simulink model "ThermalLoop_draft3"  (R2024b)
settings: Solver=VariableStepAuto  StartTime=0.0  StopTime=2600
model workspace (MAT data in the model file):
  HX_HX = 500
  Kpipes = 14
  PumpHeat = 50
  TM_pipe = 50
libraries: fl_lib x28, nesl_utility x18, SimscapeFluids_lib x18, simulink x1
(part 1 of 2)
settings Model: SimulationMode=accelerator  Creator=Matthew Whetham  LastModifiedBy=Matthew Whetham

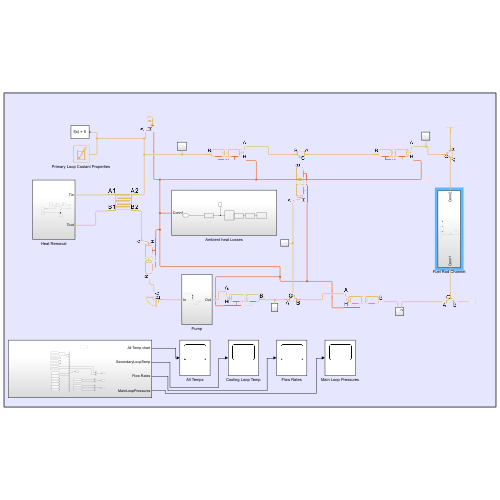
[thumbnail: Simulink's stored preview of the top-level diagram]
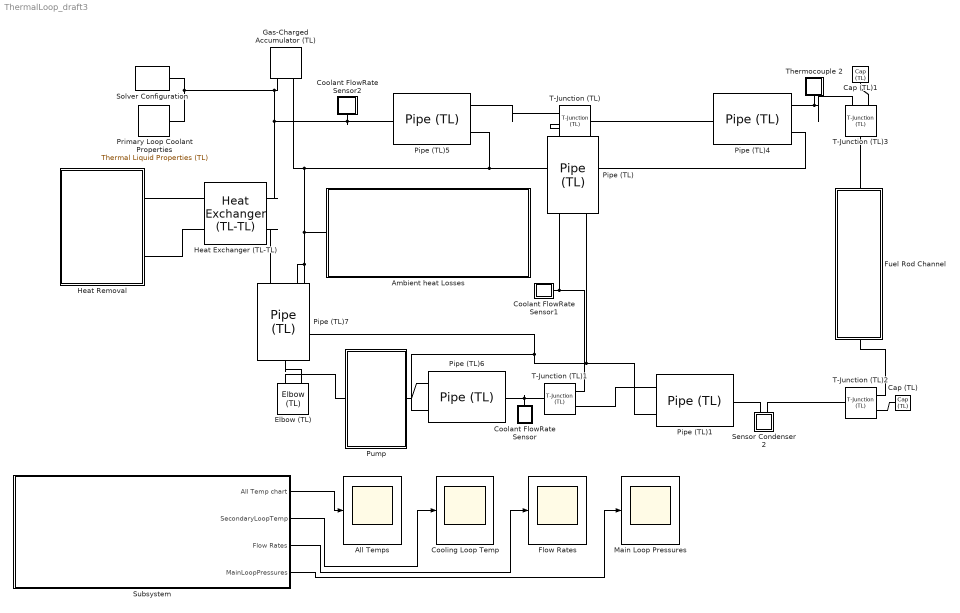
== system ThermalLoop_draft3 ==
  All Temps : Scope
  Ambient heat Losses : Subsystem
  Cap (TL) : fl_lib/Thermal Liquid/Elements/Cap (TL)  p_specify=off  p_priority=None  p=0.101325 MPa  p_nominal_specify=off  p_nominal_value=1  p_nominal_unit=MPa  T_specify=on  T_priority=Low  T=297.15 K  T_nominal_specify=off  T_nominal_value=1  T_nominal_unit=K
      settings: InternalSimscapePortConfiguration="{\"Bottom\":[],\"Left\":[{\"id\":\"A\",\"label\":\"\",\"type\":\"foundation.thermal_liquid.thermal_liquid\"}],\"Right\":[],\"Top\":[]}"
  Cap (TL)1 : fl_lib/Thermal Liquid/Elements/Cap (TL)  p_specify=off  p_priority=None  p=0.101325 MPa  p_nominal_specify=off  p_nominal_value=1  p_nominal_unit=MPa  T_specify=on  T_priority=None  T=297.15 K  T_nominal_specify=off  T_nominal_value=1  T_nominal_unit=K
      settings: InternalSimscapePortConfiguration="{\"Bottom\":[],\"Left\":[{\"id\":\"A\",\"label\":\"\",\"type\":\"foundation.thermal_liquid.thermal_liquid\"}],\"Right\":[],\"Top\":[]}"
  Coolant FlowRate Sensor : Subsystem
  Coolant FlowRate Sensor1 : Subsystem
  Coolant FlowRate Sensor2 : Subsystem
  Cooling Loop Temp : Scope
  Elbow (TL) : SimscapeFluids_lib/Thermal Liquid/Pipes & Fittings/Elbow (TL)  elbow_type=fluids.thermal_liquid.pipes_fittings.enum.ElbowType.Smooth  diameter_elbow=1.6 in  angle_elbow=90 deg  Re_c=150
      settings: InternalSimscapePortConfiguration="{\"Bottom\":[],\"Left\":[{\"id\":\"A\",\"label\":\"A\",\"type\":\"foundation.thermal_liquid.thermal_liquid\"}],\"Right\":[],\"Top\":[{\"id\":\"B\",\"label\":\"B\",\"type\":\"foundation.thermal_liquid.thermal_liquid\"}]}"
  Flow Rates : Scope
  Fuel Rod Channel : Subsystem
      settings: PortSchema="{\"entries\":[{\"content\":{\"sides\":[{\"content\":{},\"type\":\"ConnectorPlacement.EquallySpacedRectSide\",\"uuid\":\"06a059a3-807c-451a-afc8-2a90bcad8c1c\"},{\"content\":{\"side\":\"RIGHT\"},\"type\":\"ConnectorPlacement.EquallySpacedRectSide\",\"uuid\":\"c804ba08-1832-4016-bf14-7550ffa2d914\"},{\"content\":{\"connectorIds\":[\"LConn1\"],\"side\":\"TOP\"},\"type\":\"ConnectorPlacement.EquallySpacedRectSide\",\"uuid\":\"1e965a20-d254-4a65-95af-9e712761d911\"},{\"content\":{\"connectorIds\":[\"RConn1\"],\"side\":\"BOTTOM\"},\"type\":\"ConnectorPlacement.EquallySpacedRectSide\",\"uuid\":\"83471166-a379-4b82-b772-802eda07252c\"}]},\"type\":\"ConnectorPlacement.EquallySpacedConnector\",\"uuid\":\"06615f34-1427-44b4-a4dd-e60277b52231\"}],\"packageUris\":[\"http://schema.mathworks.com/mf0/Connector/R2020b\"],\"version\":\"1.0\"}"
  Gas-Charged Accumulator (TL) : SimscapeFluids_lib/Thermal Liquid/Tanks & Accumulators/Gas-Charged Accumulator (TL)  capacity=0.2 l  dead_volume=0.145 l  p_precharge_gauge=1 bar  k_sh=1.4  area=1.76 in^2  stiff_coeff=1e4 MPa/m^3  damping_coeff=1e4 MPa*s/m^6  liquid_volume_specify=off  liquid_volume_priority=High  liquid_volume=5e-3 m^3  liquid_volume_nominal_specify=off  liquid_volume_nominal_value=1  liquid_volume_nominal_unit=m^3  liquid_mass_specify=off  liquid_mass_priority=None  liquid_mass=5 kg  liquid_mass_nominal_specify=off  liquid_mass_nominal_value=1  liquid_mass_nominal_unit=kg  p_I_specify=off  p_I_priority=None  p_I=0.101325 MPa  p_I_nominal_specify=off  p_I_nominal_value=1  p_I_nominal_unit=MPa  T_I_specify=on  T_I_priority=Low  T_I=23 degC  T_I_nominal_specify=off  T_I_nominal_value=1  T_I_nominal_unit=K
      settings: InternalSimscapePortConfiguration="{\"Bottom\":[],\"Left\":[],\"Right\":[{\"id\":\"A\",\"label\":\"A\",\"type\":\"foundation.thermal_liquid.thermal_liquid\"},{\"id\":\"H\",\"label\":\"H\",\"type\":\"foundation.thermal.thermal\"}],\"Top\":[]}"
  Heat Exchanger (TL-TL) : SimscapeFluids_lib/Heat Exchangers/Thermal Liquid/Heat Exchanger (TL-TL)  hex_type=fluids.heat_exchangers.enum.FlowArrangement.ShellTube  shell_num=1  cross_type=fluids.heat_exchangers.enum.CrossFlowArrangementTLTL.MixedMixed  NTU_TLU=[.5, 1, 2, 3, 4, 5]  CR_TLU=[0, .25, .5, .75, 1]  eff_TLU=[.3, .3, .3, .3, .3; .6, .55, .5, .47, .43; .85, .76, .68, .61, .55; .94, .83, .72, .65, .58; .98, .86, .75, .66, .58; .99, .86, .75, .66, .58]  wall_thermal_dynamics=false  thermal_mass_wall=447 J/K  R_wall=1.6e-5 K/W  min_flow_area_1=1 m^2  Dh_press_1=0.1 m  liquid_volume_1=0.01 m^3  Re_lam_1=2000  Re_tur_1=4000  pressure_loss_spec_1=fluids.heat_exchangers.enum.PressureLossSpec.LossCoeff  pressure_loss_coeff_1=0.1  length_press_1=1 m  length_add_1=0.1 m  roughness_1=15e-6 m  Re_friction_TLU_1=[400, 1000, 1500, 3000, 4000, 6000, 10000, 20000, 40000, 60000, 100000, 100000000]  friction_factor_TLU_1=[.264, .112, .071, .0417, .0387, .0268, .025, .0232, .0226, .022, .0214, .0214]  shape_factor_1=64  Re_Euler_TLU_1=[50, 500, 1000, 2000]  Euler_TLU_1=[4.4505, .6864, .4791, .3755]  heat_transfer_spec_1=fluids.heat_exchangers.enum.HeatCoeffSpec.Constant  heat_transfer_area_1=1 m^2  heat_coeff_1=HX_HX W/(K*m^2)  length_heat_1=1 m  Nu_lam_1=3.66  Re_Colburn_TLU_1=[100, 150, 1000]  Colburn_factor_TLU_1=[.019, .013, .002]  Re_Nu_TLU_1=[100, 150, 1000]  Pr_Nu_TLU_1=[1, 10]  Nu_TLU_1=[3.72, 4.21; 3.75, 4.44; 4.21, 7.15]  fouling_factor_1=1e-4 K*m^2/W  min_heat_coeff_1=100 W/(K*m^2)  min_flow_area_2=1 m^2  Dh_press_2=0.1 m  liquid_volume_2=0.01 m^3  Re_lam_2=2000  Re_tur_2=4000  pressure_loss_spec_2=fluids.heat_exchangers.enum.PressureLossSpec.LossCoeff  pressure_loss_coeff_2=0.1  length_press_2=1 m  length_add_2=0.1 m  roughness_2=15e-6 m  Re_friction_TLU_2=[400, 1000, 1500, 3000, 4000, 6000, 10000, 20000, 40000, 60000, 100000, 100000000]  friction_factor_TLU_2=[.264, .112, .071, .0417, .0387, .0268, .025, .0232, .0226, .022, .0214, .0214]  shape_factor_2=64  Re_Euler_TLU_2=[50, 500, 1000, 2000]  Euler_TLU_2=[4.4505, .6864, .4791, .3755]  heat_transfer_spec_2=fluids.heat_exchangers.enum.HeatCoeffSpec.Constant  heat_transfer_area_2=1 m^2  heat_coeff_2=HX_HX W/(K*m^2)  length_heat_2=1 m  Nu_lam_2=3.66  Re_Colburn_TLU_2=[100, 150, 1000]  Colburn_factor_TLU_2=[.019, .013, .002]  Re_Nu_TLU_2=[100, 150, 1000]  Pr_Nu_TLU_2=[1, 10]  Nu_TLU_2=[3.72, 4.21; 3.75, 4.44; 4.21, 7.15]  fouling_factor_2=1e-4 K*m^2/W  min_heat_coeff_2=100 W/(K*m^2)  dynamic_compressibility_1=false  T0_1=23 degC  p0_1=0.101325 MPa  dynamic_compressibility_2=false  T0_2=23 degC  p0_2=0.101325 MPa
      settings: InternalSimscapePortConfiguration="{\"Bottom\":[],\"Left\":[{\"id\":\"A1\",\"label\":\"A1\",\"type\":\"foundation.thermal_liquid.thermal_liquid\"},{\"id\":\"B1\",\"label\":\"B1\",\"type\":\"foundation.thermal_liquid.thermal_liquid\"}],\"Right\":[{\"id\":\"A2\",\"label\":\"A2\",\"type\":\"foundation.thermal_liquid.thermal_liquid\"},{\"id\":\"B2\",\"label\":\"B2\",\"type\":\"foundation.thermal_liquid.thermal_liquid\"}],\"Top\":[]}"
  Heat Removal : Subsystem
  Main Loop Pressures : Scope
  Pipe (TL) : SimscapeFluids_lib/Thermal Liquid/Pipes & Fittings/Pipe (TL)  dynamic_compressibility=true  inertia=false  num_segments=1  pipe_length=68.75 in  cross_section_geometry=fluids.thermal_liquid.pipes_fittings.enum.CrossSectionGeometry.Circular  pipe_diameter=1.6 in  pipe_inner_diameter=0.05 m  pipe_outer_diameter=0.1 m  pipe_width=0.1 m  pipe_height=0.1 m  pipe_major_axis=0.1 m  pipe_minor_axis=0.05 m  pipe_side=0.1 m  pipe_angle=30 deg  area=0.01 m^2  Dh=0.1128 m  elevation_spec=foundation.enum.constant_variable.constant  elevation_gain=68.75 in  gravity_spec=foundation.enum.constant_variable.constant  g=9.81 m/s^2  pressure_loss_spec=fluids.thermal_liquid.pipes_fittings.enum.PressureLossSpec.Haaland  local_pressure_loss_spec=fluids.thermal_liquid.pipes_fittings.enum.LocalLossSpec.AggregateLength  length_add=1 m  loss_coefficient=0.1  roughness_spec=fluids.thermal_liquid.pipes_fittings.enum.RoughnessSpec.SteelWroughtIron  roughness=15e-6 m  Re_friction_TLU=[400, 1000, 1500, 3000, 4000, 6000, 10000, 20000, 40000, 60000, 100000, 100000000]  friction_factor_TLU=[.264, .112, .071, .0417, .0387, .0268, .025, .0232, .0226, .022, .0214, .0214]  Re_lam=2000  Re_tur=4000  shape_factor=64  mdot_nominal=[.1, 1] kg/s  p_diff_nominal=[.001, .01] MPa  mdot_threshold=1e-6 kg/s  wall_spec=fluids.thermal_liquid.pipes_fittings.enum.wall_spec.rigid  vol_expansion_spec=fluids.thermal_liquid.pipes_fittings.enum.VolumeExpansionSpec.Area  area_pressure_gain=1e-6 m^2/MPa  static_pressure_TLU=[.1, 1] MPa  area_pressure_gain_TLU=[1e-05, 1.1e-05] m^2  material_behavior_spec=fluids.thermal_liquid.pipes_fittings.enum.PipeMaterialBehavior.Linear  diameter_pressure_gain=1e-6 m/MPa  wall_thickness=0.05 m  elastic_modulus=69 GPa  stress_TLU=[276, 310] MPa  strain_TLU=[.004, .02]  stress_assert_action=simscape.enum.assert.action.none  stress_max=400 MPa  poisson_ratio=0.33  wall_time_constant=0.01 s  thermal_expansion=false  alpha_L_wall=24 um/(deltaK*m)  thermal_expansion_Tref=293.15 K  heat_transfer_spec=fluids.thermal_liquid.pipes_fittings.enum.HeatTransferSpec.Gnielinski  mdot_nominal_heat=[.1, 1] kg/s  T_in_nominal=[293.15, 293.15] K  T_out_nominal=[300, 300] K  p_in_nominal_heat=[.101325, .101325] MPa  T_wall_nominal=[303.15, 303.15] K  a_coeff=0.023  b_Re_power=0.8  c_Pr_power=0.4  Nu_lam=3.66  Re_Colburn_TLU=[100, 150, 1000]  Colburn_factor_TLU=[.019, .013, .002]  Re_Nu_TLU=[100, 150, 1000]  Pr_Nu_TLU=[1, 10]  Nu_TLU=[3.72, 4.21; 3.75, 4.44; 4.21, 7.15]  p0_vec=0.101325 MPa  T0_vec=23 degC  mdot0=0.1 kg/s
  Pipe (TL)1 : SimscapeFluids_lib/Thermal Liquid/Pipes & Fittings/Pipe (TL)  dynamic_compressibility=true  inertia=false  num_segments=1  pipe_length=155.4 in  cross_section_geometry=fluids.thermal_liquid.pipes_fittings.enum.CrossSectionGeometry.Circular  pipe_diameter=1.6 in  pipe_inner_diameter=0.05 m  pipe_outer_diameter=0.1 m  pipe_width=0.1 m  pipe_height=0.1 m  pipe_major_axis=0.1 m  pipe_minor_axis=0.05 m  pipe_side=0.1 m  pipe_angle=30 deg  area=0.01 m^2  Dh=0.1128 m  elevation_spec=foundation.enum.constant_variable.constant  elevation_gain=0 in  gravity_spec=foundation.enum.constant_variable.constant  g=9.81 m/s^2  pressure_loss_spec=fluids.thermal_liquid.pipes_fittings.enum.PressureLossSpec.Haaland  local_pressure_loss_spec=fluids.thermal_liquid.pipes_fittings.enum.LocalLossSpec.AggregateLength  length_add=1 m  loss_coefficient=0.1  roughness_spec=fluids.thermal_liquid.pipes_fittings.enum.RoughnessSpec.SteelWroughtIron  roughness=15e-6 m  Re_friction_TLU=[400, 1000, 1500, 3000, 4000, 6000, 10000, 20000, 40000, 60000, 100000, 100000000]  friction_factor_TLU=[.264, .112, .071, .0417, .0387, .0268, .025, .0232, .0226, .022, .0214, .0214]  Re_lam=2000  Re_tur=4000  shape_factor=64  mdot_nominal=[.1, 1] kg/s  p_diff_nominal=[.001, .01] MPa  mdot_threshold=1e-6 kg/s  wall_spec=fluids.thermal_liquid.pipes_fittings.enum.wall_spec.rigid  vol_expansion_spec=fluids.thermal_liquid.pipes_fittings.enum.VolumeExpansionSpec.Area  area_pressure_gain=1e-6 m^2/MPa  static_pressure_TLU=[.1, 1] MPa  area_pressure_gain_TLU=[1e-05, 1.1e-05] m^2  material_behavior_spec=fluids.thermal_liquid.pipes_fittings.enum.PipeMaterialBehavior.Linear  diameter_pressure_gain=1e-6 m/MPa  wall_thickness=0.05 m  elastic_modulus=69 GPa  stress_TLU=[276, 310] MPa  strain_TLU=[.004, .02]  stress_assert_action=simscape.enum.assert.action.none  stress_max=400 MPa  poisson_ratio=0.33  wall_time_constant=0.01 s  thermal_expansion=false  alpha_L_wall=24 um/(deltaK*m)  thermal_expansion_Tref=293.15 K  heat_transfer_spec=fluids.thermal_liquid.pipes_fittings.enum.HeatTransferSpec.Gnielinski  mdot_nominal_heat=[.1, 1] kg/s  T_in_nominal=[293.15, 293.15] K  T_out_nominal=[300, 300] K  p_in_nominal_heat=[.101325, .101325] MPa  T_wall_nominal=[303.15, 303.15] K  a_coeff=0.023  b_Re_power=0.8  c_Pr_power=0.4  Nu_lam=3.66  Re_Colburn_TLU=[100, 150, 1000]  Colburn_factor_TLU=[.019, .013, .002]  Re_Nu_TLU=[100, 150, 1000]  Pr_Nu_TLU=[1, 10]  Nu_TLU=[3.72, 4.21; 3.75, 4.44; 4.21, 7.15]  p0_vec=0.101325 MPa  T0_vec=23 degC  mdot0=0.1 kg/s
  Pipe (TL)4 : SimscapeFluids_lib/Thermal Liquid/Pipes & Fittings/Pipe (TL)  dynamic_compressibility=true  inertia=false  num_segments=1  pipe_length=55.4 in  cross_section_geometry=fluids.thermal_liquid.pipes_fittings.enum.CrossSectionGeometry.Circular  pipe_diameter=1.6 in  pipe_inner_diameter=0.05 m  pipe_outer_diameter=0.1 m  pipe_width=0.1 m  pipe_height=0.1 m  pipe_major_axis=0.1 m  pipe_minor_axis=0.05 m  pipe_side=0.1 m  pipe_angle=30 deg  area=0.01 m^2  Dh=0.1128 m  elevation_spec=foundation.enum.constant_variable.constant  elevation_gain=0 in  gravity_spec=foundation.enum.constant_variable.constant  g=9.81 m/s^2  pressure_loss_spec=fluids.thermal_liquid.pipes_fittings.enum.PressureLossSpec.Haaland  local_pressure_loss_spec=fluids.thermal_liquid.pipes_fittings.enum.LocalLossSpec.AggregateLength  length_add=1 m  loss_coefficient=0.1  roughness_spec=fluids.thermal_liquid.pipes_fittings.enum.RoughnessSpec.SteelWroughtIron  roughness=15e-6 m  Re_friction_TLU=[400, 1000, 1500, 3000, 4000, 6000, 10000, 20000, 40000, 60000, 100000, 100000000]  friction_factor_TLU=[.264, .112, .071, .0417, .0387, .0268, .025, .0232, .0226, .022, .0214, .0214]  Re_lam=2000  Re_tur=4000  shape_factor=64  mdot_nominal=[.1, 1] kg/s  p_diff_nominal=[.001, .01] MPa  mdot_threshold=1e-6 kg/s  wall_spec=fluids.thermal_liquid.pipes_fittings.enum.wall_spec.rigid  vol_expansion_spec=fluids.thermal_liquid.pipes_fittings.enum.VolumeExpansionSpec.Area  area_pressure_gain=1e-6 m^2/MPa  static_pressure_TLU=[.1, 1] MPa  area_pressure_gain_TLU=[1e-05, 1.1e-05] m^2  material_behavior_spec=fluids.thermal_liquid.pipes_fittings.enum.PipeMaterialBehavior.Linear  diameter_pressure_gain=1e-6 m/MPa  wall_thickness=0.05 m  elastic_modulus=69 GPa  stress_TLU=[276, 310] MPa  strain_TLU=[.004, .02]  stress_assert_action=simscape.enum.assert.action.none  stress_max=400 MPa  poisson_ratio=0.33  wall_time_constant=0.01 s  thermal_expansion=false  alpha_L_wall=24 um/(deltaK*m)  thermal_expansion_Tref=293.15 K  heat_transfer_spec=fluids.thermal_liquid.pipes_fittings.enum.HeatTransferSpec.Gnielinski  mdot_nominal_heat=[.1, 1] kg/s  T_in_nominal=[293.15, 293.15] K  T_out_nominal=[300, 300] K  p_in_nominal_heat=[.101325, .101325] MPa  T_wall_nominal=[303.15, 303.15] K  a_coeff=0.023  b_Re_power=0.8  c_Pr_power=0.4  Nu_lam=3.66  Re_Colburn_TLU=[100, 150, 1000]  Colburn_factor_TLU=[.019, .013, .002]  Re_Nu_TLU=[100, 150, 1000]  Pr_Nu_TLU=[1, 10]  Nu_TLU=[3.72, 4.21; 3.75, 4.44; 4.21, 7.15]  p0_vec=0.101325 MPa  T0_vec=23 degC  mdot0=0.1 kg/s
  Pipe (TL)5 : SimscapeFluids_lib/Thermal Liquid/Pipes & Fittings/Pipe (TL)  dynamic_compressibility=true  inertia=false  num_segments=1  pipe_length=57.45 in  cross_section_geometry=fluids.thermal_liquid.pipes_fittings.enum.CrossSectionGeometry.Circular  pipe_diameter=1.6 in  pipe_inner_diameter=0.05 m  pipe_outer_diameter=0.1 m  pipe_width=0.1 m  pipe_height=0.1 m  pipe_major_axis=0.1 m  pipe_minor_axis=0.05 m  pipe_side=0.1 m  pipe_angle=30 deg  area=0.01 m^2  Dh=0.1128 m  elevation_spec=foundation.enum.constant_variable.constant  elevation_gain=0 m  gravity_spec=foundation.enum.constant_variable.constant  g=9.81 m/s^2  pressure_loss_spec=fluids.thermal_liquid.pipes_fittings.enum.PressureLossSpec.Haaland  local_pressure_loss_spec=fluids.thermal_liquid.pipes_fittings.enum.LocalLossSpec.AggregateLength  length_add=1 m  loss_coefficient=0.1  roughness_spec=fluids.thermal_liquid.pipes_fittings.enum.RoughnessSpec.SteelWroughtIron  roughness=15e-6 m  Re_friction_TLU=[400, 1000, 1500, 3000, 4000, 6000, 10000, 20000, 40000, 60000, 100000, 100000000]  friction_factor_TLU=[.264, .112, .071, .0417, .0387, .0268, .025, .0232, .0226, .022, .0214, .0214]  Re_lam=2000  Re_tur=4000  shape_factor=64  mdot_nominal=[.1, 1] kg/s  p_diff_nominal=[.001, .01] MPa  mdot_threshold=1e-6 kg/s  wall_spec=fluids.thermal_liquid.pipes_fittings.enum.wall_spec.rigid  vol_expansion_spec=fluids.thermal_liquid.pipes_fittings.enum.VolumeExpansionSpec.Area  area_pressure_gain=1e-6 m^2/MPa  static_pressure_TLU=[.1, 1] MPa  area_pressure_gain_TLU=[1e-05, 1.1e-05] m^2  material_behavior_spec=fluids.thermal_liquid.pipes_fittings.enum.PipeMaterialBehavior.Linear  diameter_pressure_gain=1e-6 m/MPa  wall_thickness=0.05 m  elastic_modulus=69 GPa  stress_TLU=[276, 310] MPa  strain_TLU=[.004, .02]  stress_assert_action=simscape.enum.assert.action.none  stress_max=400 MPa  poisson_ratio=0.33  wall_time_constant=0.01 s  thermal_expansion=false  alpha_L_wall=24 um/(deltaK*m)  thermal_expansion_Tref=293.15 K  heat_transfer_spec=fluids.thermal_liquid.pipes_fittings.enum.HeatTransferSpec.Gnielinski  mdot_nominal_heat=[.1, 1] kg/s  T_in_nominal=[293.15, 293.15] K  T_out_nominal=[300, 300] K  p_in_nominal_heat=[.101325, .101325] MPa  T_wall_nominal=[303.15, 303.15] K  a_coeff=0.023  b_Re_power=0.8  c_Pr_power=0.4  Nu_lam=3.66  Re_Colburn_TLU=[100, 150, 1000]  Colburn_factor_TLU=[.019, .013, .002]  Re_Nu_TLU=[100, 150, 1000]  Pr_Nu_TLU=[1, 10]  Nu_TLU=[3.72, 4.21; 3.75, 4.44; 4.21, 7.15]  p0_vec=0.101325 MPa  T0_vec=23 degC  mdot0=0.1 kg/s
  Pipe (TL)6 : SimscapeFluids_lib/Thermal Liquid/Pipes & Fittings/Pipe (TL)  dynamic_compressibility=true  inertia=false  num_segments=1  pipe_length=57.45 in  cross_section_geometry=fluids.thermal_liquid.pipes_fittings.enum.CrossSectionGeometry.Circular  pipe_diameter=1.6 in  pipe_inner_diameter=0.05 m  pipe_outer_diameter=0.1 m  pipe_width=0.1 m  pipe_height=0.1 m  pipe_major_axis=0.1 m  pipe_minor_axis=0.05 m  pipe_side=0.1 m  pipe_angle=30 deg  area=0.01 m^2  Dh=0.1128 m  elevation_spec=foundation.enum.constant_variable.constant  elevation_gain=0 m  gravity_spec=foundation.enum.constant_variable.constant  g=9.81 m/s^2  pressure_loss_spec=fluids.thermal_liquid.pipes_fittings.enum.PressureLossSpec.Haaland  local_pressure_loss_spec=fluids.thermal_liquid.pipes_fittings.enum.LocalLossSpec.AggregateLength  length_add=1 m  loss_coefficient=0.1  roughness_spec=fluids.thermal_liquid.pipes_fittings.enum.RoughnessSpec.SteelWroughtIron  roughness=15e-6 m  Re_friction_TLU=[400, 1000, 1500, 3000, 4000, 6000, 10000, 20000, 40000, 60000, 100000, 100000000]  friction_factor_TLU=[.264, .112, .071, .0417, .0387, .0268, .025, .0232, .0226, .022, .0214, .0214]  Re_lam=2000  Re_tur=4000  shape_factor=64  mdot_nominal=[.1, 1] kg/s  p_diff_nominal=[.001, .01] MPa  mdot_threshold=1e-6 kg/s  wall_spec=fluids.thermal_liquid.pipes_fittings.enum.wall_spec.rigid  vol_expansion_spec=fluids.thermal_liquid.pipes_fittings.enum.VolumeExpansionSpec.Area  area_pressure_gain=1e-6 m^2/MPa  static_pressure_TLU=[.1, 1] MPa  area_pressure_gain_TLU=[1e-05, 1.1e-05] m^2  material_behavior_spec=fluids.thermal_liquid.pipes_fittings.enum.PipeMaterialBehavior.Linear  diameter_pressure_gain=1e-6 m/MPa  wall_thickness=0.05 m  elastic_modulus=69 GPa  stress_TLU=[276, 310] MPa  strain_TLU=[.004, .02]  stress_assert_action=simscape.enum.assert.action.none  stress_max=400 MPa  poisson_ratio=0.33  wall_time_constant=0.01 s  thermal_expansion=false  alpha_L_wall=24 um/(deltaK*m)  thermal_expansion_Tref=293.15 K  heat_transfer_spec=fluids.thermal_liquid.pipes_fittings.enum.HeatTransferSpec.Gnielinski  mdot_nominal_heat=[.1, 1] kg/s  T_in_nominal=[293.15, 293.15] K  T_out_nominal=[300, 300] K  p_in_nominal_heat=[.101325, .101325] MPa  T_wall_nominal=[303.15, 303.15] K  a_coeff=0.023  b_Re_power=0.8  c_Pr_power=0.4  Nu_lam=3.66  Re_Colburn_TLU=[100, 150, 1000]  Colburn_factor_TLU=[.019, .013, .002]  Re_Nu_TLU=[100, 150, 1000]  Pr_Nu_TLU=[1, 10]  Nu_TLU=[3.72, 4.21; 3.75, 4.44; 4.21, 7.15]  p0_vec=0.101325 MPa  T0_vec=23 degC  mdot0=0.1 kg/s
  Pipe (TL)7 : SimscapeFluids_lib/Thermal Liquid/Pipes & Fittings/Pipe (TL)  dynamic_compressibility=true  inertia=false  num_segments=1  pipe_length=68.75 in  cross_section_geometry=fluids.thermal_liquid.pipes_fittings.enum.CrossSectionGeometry.Circular  pipe_diameter=1.6 in  pipe_inner_diameter=0.05 m  pipe_outer_diameter=0.1 m  pipe_width=0.1 m  pipe_height=0.1 m  pipe_major_axis=0.1 m  pipe_minor_axis=0.05 m  pipe_side=0.1 m  pipe_angle=30 deg  area=0.01 m^2  Dh=0.1128 m  elevation_spec=foundation.enum.constant_variable.constant  elevation_gain=-68.75 in  gravity_spec=foundation.enum.constant_variable.constant  g=9.81 m/s^2  pressure_loss_spec=fluids.thermal_liquid.pipes_fittings.enum.PressureLossSpec.Haaland  local_pressure_loss_spec=fluids.thermal_liquid.pipes_fittings.enum.LocalLossSpec.AggregateLength  length_add=1 m  loss_coefficient=0.1  roughness_spec=fluids.thermal_liquid.pipes_fittings.enum.RoughnessSpec.SteelWroughtIron  roughness=15e-6 m  Re_friction_TLU=[400, 1000, 1500, 3000, 4000, 6000, 10000, 20000, 40000, 60000, 100000, 100000000]  friction_factor_TLU=[.264, .112, .071, .0417, .0387, .0268, .025, .0232, .0226, .022, .0214, .0214]  Re_lam=2000  Re_tur=4000  shape_factor=64  mdot_nominal=[.1, 1] kg/s  p_diff_nominal=[.001, .01] MPa  mdot_threshold=1e-6 kg/s  wall_spec=fluids.thermal_liquid.pipes_fittings.enum.wall_spec.rigid  vol_expansion_spec=fluids.thermal_liquid.pipes_fittings.enum.VolumeExpansionSpec.Area  area_pressure_gain=1e-6 m^2/MPa  static_pressure_TLU=[.1, 1] MPa  area_pressure_gain_TLU=[1e-05, 1.1e-05] m^2  material_behavior_spec=fluids.thermal_liquid.pipes_fittings.enum.PipeMaterialBehavior.Linear  diameter_pressure_gain=1e-6 m/MPa  wall_thickness=0.05 m  elastic_modulus=69 GPa  stress_TLU=[276, 310] MPa  strain_TLU=[.004, .02]  stress_assert_action=simscape.enum.assert.action.none  stress_max=400 MPa  poisson_ratio=0.33  wall_time_constant=0.01 s  thermal_expansion=false  alpha_L_wall=24 um/(deltaK*m)  thermal_expansion_Tref=293.15 K  heat_transfer_spec=fluids.thermal_liquid.pipes_fittings.enum.HeatTransferSpec.Gnielinski  mdot_nominal_heat=[.1, 1] kg/s  T_in_nominal=[293.15, 293.15] K  T_out_nominal=[300, 300] K  p_in_nominal_heat=[.101325, .101325] MPa  T_wall_nominal=[303.15, 303.15] K  a_coeff=0.023  b_Re_power=0.8  c_Pr_power=0.4  Nu_lam=3.66  Re_Colburn_TLU=[100, 150, 1000]  Colburn_factor_TLU=[.019, .013, .002]  Re_Nu_TLU=[100, 150, 1000]  Pr_Nu_TLU=[1, 10]  Nu_TLU=[3.72, 4.21; 3.75, 4.44; 4.21, 7.15]  p0_vec=0.101325 MPa  T0_vec=23 degC  mdot0=0.1 kg/s
  Primary Loop Coolant Properties : SimscapeFluids_lib/Thermal Liquid/Utilities/Thermal Liquid Properties (TL)  fluid_list=fluids.thermal_liquid.utilities.enum.thermal_liquid_fluid_list.water  concentration_param_EG=fluids.thermal_liquid.utilities.enum.thermal_liquid_concentration.volume_fraction  concentration_param_PG=fluids.thermal_liquid.utilities.enum.thermal_liquid_concentration.volume_fraction  c_mass_SW=3.5e-3  c_mass_EG=0.1  c_mass_PG=0.1  c_mass_GL=0.1  c_vol_EG=0.1  c_vol_PG=0.1  beta_const_EG=2.1791 GPa  beta_const_PG=2.1791 GPa  beta_const_GL=2.1791 GPa  p_min_EG=0.01 MPa  p_min_PG=0.01 MPa  p_min_GL=0.01 MPa  p_max_EG=50 MPa  p_max_PG=50 MPa  p_max_GL=50 MPa  p_atm=0.101325 MPa  properties_range_check=simscape.enum.assert.action.none
  Pump : Subsystem
  Sensor Condenser 2 : Subsystem
  Solver Configuration : nesl_utility/Solver Configuration  PhysicalDomain=network_engine_domain  SubClassName=solver  LeftPortType=input  RightPortType=generic  Tones=[]  Harmonics=[]  SimulateNoise=off  Profile=off  UseLocalSampling=off  EnableSwitchedLinearOptims=on  FrequencyDomain=off  UseCCode=off  RelTol=0.001  AbsTol=0.001  MinStep=1e-09  ToWorkspace=off  RevertToSquareIcSolve=off  NumHomotopyIterations=100  PhasorMode=off  PhasorModeNumHarmonics=1  ConsistencySolver=NEWTON_XTOL_AFTER_FTOL  IndexReductionMethod=DerivativeReplacement  DoDC=on  ResidualTolerance=1e-09  ConsistencyTolSource=GLOBAL  ConsistencyAbsTol=0.001  ConsistencyRelTol=0.001  ConsistencyTolFactor=0.001  UseLocalSolver=off  LocalSolverChoice=NE_BACKWARD_EULER_ADVANCER  ResolveIndetEquations=on  FunctionEvalNumThread=1  LocalSolverSampleTime=0.001  DoFixedCost=off  MaxNonlinIter=3  MaxModeIter=2  ComputeImpulses=off  ImpulseIterations=2  LinearAlgebra=auto  LinearAlgebraNumThread=0  EquationFormulation=NE_TIME_EF  DelaysMemoryBudget=1024  AutomaticFiltering=on  FilteringTimeConstant=0.001  PartitionStorageMethod=AS_NEEDED  PartitionMemoryBudget=1024  PartitionMethod=ROBUST  MultibodyUseLocalSolver=off  MultibodyLocalSolverChoice=ODE1  MultibodyLocalSolverSampleTime=0.001
  Subsystem : Subsystem
  T-Junction (TL){,1..3} (4 alike) : SimscapeFluids_lib/Thermal Liquid/Pipes & Fittings/T-Junction (TL)  area_main=1.6 in^2  area_branch=1.6 in^2  junction_spec=fluids.thermal_liquid.pipes_fittings.enum.TLossCoefficientModel.Crane  k_main_converge=1.12  k_main_diverge=1.12  k_branch_converge=1.12  k_branch_diverge=1.12  loss_coeff_A=1  loss_coeff_B=1  loss_coeff_C=1  radius=0.001 m  Re_c=150  Re_0=10  tau=0.0001 s  saturation_ratio=0.2  smoothing_factor=0.01  inertia=false
      settings: InternalSimscapePortConfiguration="{\"Bottom\":[{\"id\":\"C\",\"label\":\"C\",\"type\":\"foundation.thermal_liquid.thermal_liquid\"}],\"Left\":[{\"id\":\"A\",\"label\":\"A\",\"type\":\"foundation.thermal_liquid.thermal_liquid\"}],\"Right\":[{\"id\":\"B\",\"label\":\"B\",\"type\":\"foundation.thermal_liquid.thermal_liquid\"}],\"Top\":[]}"
  Thermocouple 2 : Subsystem
  wires:
  Subsystem/1(All Temp chart) -> All Temps/1
  Subsystem/2(SecondaryLoopTemp) -> Cooling Loop Temp/1
  Subsystem/3(Flow Rates) -> Flow Rates/1
  Subsystem/4(MainLoopPressures) -> Main Loop Pressures/1
  connections:
  T-Junction (TL)1/RConn1 -- Pipe (TL)1/LConn1
  T-Junction (TL)2/RConn1 -- Cap (TL)/LConn1
  T-Junction (TL)3/RConn1 -- Cap (TL)1/LConn1
  Pipe (TL)4/LConn1 -- T-Junction (TL)3/RConn2 -- Thermocouple 2/LConn1
  Gas-Charged Accumulator (TL)/RConn1 -- Coolant FlowRate Sensor2/LConn1 -- Pipe (TL)5/RConn1 -- Heat Exchanger (TL-TL)/RConn1 -- Solver Configuration/RConn1 -- Primary Loop Coolant Properties/RConn1
  Pipe (TL)7/RConn1 -- Elbow (TL)/LConn1
  Sensor Condenser 2/LConn1 -- Pipe (TL)1/RConn1
  Pipe (TL)5/LConn1 -- T-Junction (TL)/RConn1
  Sensor Condenser 2/LConn2 -- T-Junction (TL)2/LConn1
  Pipe (TL)4/LConn2 -- Pipe (TL)5/LConn2 -- Gas-Charged Accumulator (TL)/RConn2 -- Pipe (TL)1/LConn2 -- Pipe (TL)/LConn2 -- Pipe (TL)6/LConn2 -- Pipe (TL)7/LConn2 -- Ambient heat Losses/LConn1
  T-Junction (TL)3/LConn1 -- Fuel Rod Channel/LConn1
  Fuel Rod Channel/RConn1 -- T-Junction (TL)2/RConn2
  Heat Removal/RConn1 -- Heat Exchanger (TL-TL)/LConn1
  Heat Exchanger (TL-TL)/LConn2 -- Heat Removal/RConn2
  Pump/LConn1 -- Elbow (TL)/LConn2
  Heat Exchanger (TL-TL)/RConn2 -- Pipe (TL)7/LConn1
  Pipe (TL)6/LConn1 -- Pump/RConn1
  T-Junction (TL)/LConn1 -- Pipe (TL)4/RConn1
  T-Junction (TL)1/LConn1 -- Pipe (TL)6/RConn1 -- Coolant FlowRate Sensor/LConn1
  Pipe (TL)/RConn1 -- T-Junction (TL)/RConn2
  Pipe (TL)/LConn1 -- T-Junction (TL)1/RConn2 -- Coolant FlowRate Sensor1/LConn1

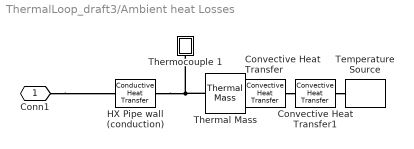
== system ThermalLoop_draft3/Ambient heat Losses ==
  Convective Heat Transfer : fl_lib/Thermal/Thermal Elements/Convective Heat Transfer  thermal_type=foundation.enum.constant_variable.constant  area=3110 in^2  heat_tr_coeff=16 W/(K*m^2)  min_heat_tr_coeff=1e-3 W/(K*m^2)  T_specify=off  T_priority=None  T=0 K  T_nominal_specify=off  T_nominal_value=1  T_nominal_unit=K  Q_specify=off  Q_priority=None  Q=0 W  Q_nominal_specify=off  Q_nominal_value=1  Q_nominal_unit=W
  Convective Heat Transfer1 : fl_lib/Thermal/Thermal Elements/Convective Heat Transfer  thermal_type=foundation.enum.constant_variable.constant  area=134088 in^2  heat_tr_coeff=12 W/(K*m^2)  min_heat_tr_coeff=1e-3 W/(K*m^2)  T_specify=off  T_priority=None  T=0 K  T_nominal_specify=off  T_nominal_value=1  T_nominal_unit=K  Q_specify=off  Q_priority=None  Q=0 W  Q_nominal_specify=off  Q_nominal_value=1  Q_nominal_unit=W
  HX Pipe wall (conduction) : fl_lib/Thermal/Thermal Elements/Conductive Heat Transfer  thermal_type=foundation.enum.ConstantVariableTabulated.Constant  wall_geometry=foundation.enum.ConductionWallGeometry.Cylindrical  area=10 in^2  thickness=4 mm  d_in=1.6 in  d_out=1.95 in  L=85 in  th_cond_min=10 W/(K*m)  th_cond=Kpipes W/(K*m)  th_cond_TLU=[413, 401, 392, 383, 371, 357, 342] W/(K*m)  temp_TLU=[200, 273, 400, 600, 800, 1000, 1200] K  T_specify=off  T_priority=None  T=0 K  T_nominal_specify=off  T_nominal_value=1  T_nominal_unit=K  Q_specify=off  Q_priority=None  Q=0 W  Q_nominal_specify=off  Q_nominal_value=1  Q_nominal_unit=W
  Temperature Source : fl_lib/Thermal/Thermal Sources/Temperature Source  temperature=23 degC
  Thermal Mass : fl_lib/Thermal/Thermal Elements/Thermal Mass  mass_type=foundation.enum.constant_variable.constant  mass=TM_pipe kg  sp_heat=1005 J/(K*kg)  mass_min=1e-6 kg  num_ports=foundation.enum.numPorts2.two  m_specify=off  m_priority=High  m=1 kg  m_nominal_specify=off  m_nominal_value=1  m_nominal_unit=kg  T_specify=on  T_priority=Low  T=297.15 K  T_nominal_specify=off  T_nominal_value=1  T_nominal_unit=K  Q_specify=off  Q_priority=None  Q=0 W  Q_nominal_specify=off  Q_nominal_value=1  Q_nominal_unit=W
      settings: InternalSimscapePortConfiguration="{\"Bottom\":[],\"Left\":[{\"id\":\"M\",\"label\":\"\",\"type\":\"foundation.thermal.thermal\"}],\"Right\":[{\"id\":\"N\",\"label\":\"\",\"type\":\"foundation.thermal.thermal\"}],\"Top\":[]}"
  Thermocouple 1 : Subsystem
  Conn1 : PMIOPort  Side=Left
  connections:
  HX Pipe wall (conduction)/RConn1 -- Thermocouple 1/LConn1 -- Thermal Mass/RConn1
  Convective Heat Transfer/RConn1 -- Convective Heat Transfer1/LConn1
  Convective Heat Transfer1/RConn1 -- Temperature Source/LConn1
  Conn1/RConn1 -- HX Pipe wall (conduction)/LConn1
  Thermal Mass/LConn1 -- Convective Heat Transfer/LConn1

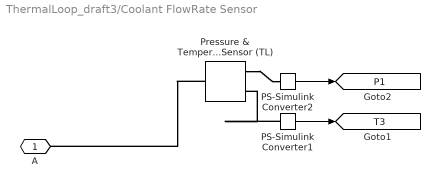
== system ThermalLoop_draft3/Coolant FlowRate Sensor ==
  PS-Simulink Converter1 : nesl_utility/PS-Simulink Converter  PhysicalDomain=network_engine_domain  SubClassName=ps_output  LeftPortType=input  RightPortType=output  PseudoPeriodic=off  Frequencies=[]  VectorFormat=inherit  Unit=degC  AffineConversion=on
  PS-Simulink Converter2 : nesl_utility/PS-Simulink Converter  PhysicalDomain=network_engine_domain  SubClassName=ps_output  LeftPortType=input  RightPortType=output  PseudoPeriodic=off  Frequencies=[]  VectorFormat=inherit  Unit=Pa  AffineConversion=on
  Pressure & Temperature Sensor (TL) : fl_lib/Thermal Liquid/Sensors/Pressure & Temperature Sensor (TL)  reference=foundation.enum.MeasurementReference.absolute  pressure=true  pressure_spec=foundation.enum.PressureMeasementSpec.Absolute  temperature=true
      settings: InternalSimscapePortConfiguration="{\"Bottom\":[{\"id\":\"T\",\"label\":\"T\",\"type\":\"output\"}],\"Left\":[{\"id\":\"A\",\"label\":\"A\",\"type\":\"foundation.thermal_liquid.thermal_liquid\"}],\"Right\":[{\"id\":\"Pa\",\"label\":\"Pa\",\"type\":\"output\"}],\"Top\":[]}"
  A : PMIOPort  Side=Left
  tag scope: P1=global, T3=global
  wires:
  PS-Simulink Converter1/1 -> [T3]
  PS-Simulink Converter2/1 -> [P1]
  connections:
  Pressure & Temperature Sensor (TL)/LConn1 -- A/RConn1
  PS-Simulink Converter1/LConn1 -- Pressure & Temperature Sensor (TL)/RConn2
  Pressure & Temperature Sensor (TL)/RConn1 -- PS-Simulink Converter2/LConn1

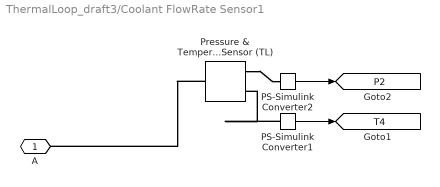
== system ThermalLoop_draft3/Coolant FlowRate Sensor1 ==
  PS-Simulink Converter1 : nesl_utility/PS-Simulink Converter  PhysicalDomain=network_engine_domain  SubClassName=ps_output  LeftPortType=input  RightPortType=output  PseudoPeriodic=off  Frequencies=[]  VectorFormat=inherit  Unit=degC  AffineConversion=on
  PS-Simulink Converter2 : nesl_utility/PS-Simulink Converter  PhysicalDomain=network_engine_domain  SubClassName=ps_output  LeftPortType=input  RightPortType=output  PseudoPeriodic=off  Frequencies=[]  VectorFormat=inherit  Unit=Pa  AffineConversion=on
  Pressure & Temperature Sensor (TL) : fl_lib/Thermal Liquid/Sensors/Pressure & Temperature Sensor (TL)  reference=foundation.enum.MeasurementReference.absolute  pressure=true  pressure_spec=foundation.enum.PressureMeasementSpec.Absolute  temperature=true
      settings: InternalSimscapePortConfiguration="{\"Bottom\":[{\"id\":\"T\",\"label\":\"T\",\"type\":\"output\"}],\"Left\":[{\"id\":\"A\",\"label\":\"A\",\"type\":\"foundation.thermal_liquid.thermal_liquid\"}],\"Right\":[{\"id\":\"Pa\",\"label\":\"Pa\",\"type\":\"output\"}],\"Top\":[]}"
  A : PMIOPort  Side=Left
  tag scope: P2=global, T4=global
  wires:
  PS-Simulink Converter1/1 -> [T4]
  PS-Simulink Converter2/1 -> [P2]
  connections:
  Pressure & Temperature Sensor (TL)/LConn1 -- A/RConn1
  PS-Simulink Converter1/LConn1 -- Pressure & Temperature Sensor (TL)/RConn2
  Pressure & Temperature Sensor (TL)/RConn1 -- PS-Simulink Converter2/LConn1

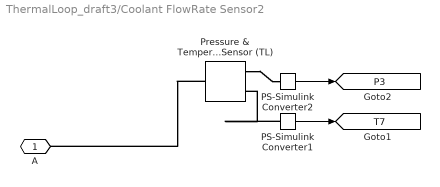
== system ThermalLoop_draft3/Coolant FlowRate Sensor2 ==
  PS-Simulink Converter1 : nesl_utility/PS-Simulink Converter  PhysicalDomain=network_engine_domain  SubClassName=ps_output  LeftPortType=input  RightPortType=output  PseudoPeriodic=off  Frequencies=[]  VectorFormat=inherit  Unit=degC  AffineConversion=on
  PS-Simulink Converter2 : nesl_utility/PS-Simulink Converter  PhysicalDomain=network_engine_domain  SubClassName=ps_output  LeftPortType=input  RightPortType=output  PseudoPeriodic=off  Frequencies=[]  VectorFormat=inherit  Unit=Pa  AffineConversion=on
  Pressure & Temperature Sensor (TL) : fl_lib/Thermal Liquid/Sensors/Pressure & Temperature Sensor (TL)  reference=foundation.enum.MeasurementReference.absolute  pressure=true  pressure_spec=foundation.enum.PressureMeasementSpec.Absolute  temperature=true
      settings: InternalSimscapePortConfiguration="{\"Bottom\":[{\"id\":\"T\",\"label\":\"T\",\"type\":\"output\"}],\"Left\":[{\"id\":\"A\",\"label\":\"A\",\"type\":\"foundation.thermal_liquid.thermal_liquid\"}],\"Right\":[{\"id\":\"Pa\",\"label\":\"Pa\",\"type\":\"output\"}],\"Top\":[]}"
  A : PMIOPort  Side=Left
  tag scope: P3=global, T7=global
  wires:
  PS-Simulink Converter1/1 -> [T7]
  PS-Simulink Converter2/1 -> [P3]
  connections:
  Pressure & Temperature Sensor (TL)/LConn1 -- A/RConn1
  PS-Simulink Converter1/LConn1 -- Pressure & Temperature Sensor (TL)/RConn2
  Pressure & Temperature Sensor (TL)/RConn1 -- PS-Simulink Converter2/LConn1

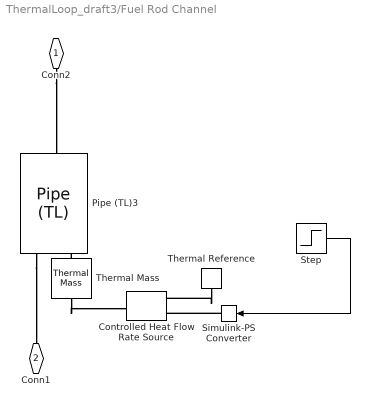
== system ThermalLoop_draft3/Fuel Rod Channel ==
  Controlled Heat Flow Rate Source : fl_lib/Thermal/Thermal Sources/Controlled Heat Flow Rate Source
  Pipe (TL)3 : SimscapeFluids_lib/Thermal Liquid/Pipes & Fittings/Pipe (TL)  dynamic_compressibility=true  inertia=false  num_segments=1  pipe_length=68.75 in  cross_section_geometry=fluids.thermal_liquid.pipes_fittings.enum.CrossSectionGeometry.Circular  pipe_diameter=1.6 in  pipe_inner_diameter=0.05 m  pipe_outer_diameter=0.1 m  pipe_width=0.1 m  pipe_height=0.1 m  pipe_major_axis=0.1 m  pipe_minor_axis=0.05 m  pipe_side=0.1 m  pipe_angle=30 deg  area=0.01 m^2  Dh=0.1128 m  elevation_spec=foundation.enum.constant_variable.constant  elevation_gain=68.75 in  gravity_spec=foundation.enum.constant_variable.constant  g=9.81 m/s^2  pressure_loss_spec=fluids.thermal_liquid.pipes_fittings.enum.PressureLossSpec.Haaland  local_pressure_loss_spec=fluids.thermal_liquid.pipes_fittings.enum.LocalLossSpec.AggregateLength  length_add=1 m  loss_coefficient=0.1  roughness_spec=fluids.thermal_liquid.pipes_fittings.enum.RoughnessSpec.CommercialPipe  roughness=15e-6 m  Re_friction_TLU=[400, 1000, 1500, 3000, 4000, 6000, 10000, 20000, 40000, 60000, 100000, 100000000]  friction_factor_TLU=[.264, .112, .071, .0417, .0387, .0268, .025, .0232, .0226, .022, .0214, .0214]  Re_lam=2000  Re_tur=4000  shape_factor=64  mdot_nominal=[.1, 1] kg/s  p_diff_nominal=[.001, .01] MPa  mdot_threshold=1e-6 kg/s  wall_spec=fluids.thermal_liquid.pipes_fittings.enum.wall_spec.rigid  vol_expansion_spec=fluids.thermal_liquid.pipes_fittings.enum.VolumeExpansionSpec.Area  area_pressure_gain=1e-6 m^2/MPa  static_pressure_TLU=[.1, 1] MPa  area_pressure_gain_TLU=[1e-05, 1.1e-05] m^2  material_behavior_spec=fluids.thermal_liquid.pipes_fittings.enum.PipeMaterialBehavior.Linear  diameter_pressure_gain=1e-6 m/MPa  wall_thickness=0.05 m  elastic_modulus=69 GPa  stress_TLU=[276, 310] MPa  strain_TLU=[.004, .02]  stress_assert_action=simscape.enum.assert.action.none  stress_max=400 MPa  poisson_ratio=0.33  wall_time_constant=0.01 s  thermal_expansion=false  alpha_L_wall=24 um/(deltaK*m)  thermal_expansion_Tref=293.15 K  heat_transfer_spec=fluids.thermal_liquid.pipes_fittings.enum.HeatTransferSpec.Gnielinski  mdot_nominal_heat=[.1, 1] kg/s  T_in_nominal=[293.15, 293.15] K  T_out_nominal=[300, 300] K  p_in_nominal_heat=[.101325, .101325] MPa  T_wall_nominal=[303.15, 303.15] K  a_coeff=0.023  b_Re_power=0.8  c_Pr_power=0.4  Nu_lam=3.66  Re_Colburn_TLU=[100, 150, 1000]  Colburn_factor_TLU=[.019, .013, .002]  Re_Nu_TLU=[100, 150, 1000]  Pr_Nu_TLU=[1, 10]  Nu_TLU=[3.72, 4.21; 3.75, 4.44; 4.21, 7.15]  p0_vec=0.101325 MPa  T0_vec=23 degC  mdot0=0.1 kg/s
  Simulink-PS Converter : nesl_utility/Simulink-PS Converter  PhysicalDomain=network_engine_domain  SubClassName=ps_input  LeftPortType=input  RightPortType=output  PseudoPeriodic=off  Frequencies=[]  NoiseDistribution=none  NoiseParameters=[]  Unit=W  AffineConversion=off  FilteringAndDerivatives=provide  SimscapeFilterOrder=1  InputFilterTimeConstant=0.001  UdotUserProvided=0
  Step : Step  After=240  SampleTime=0
  Thermal Mass : fl_lib/Thermal/Thermal Elements/Thermal Mass  mass_type=foundation.enum.constant_variable.constant  mass=3 kg  sp_heat=447 J/(K*kg)  mass_min=1e-6 kg  num_ports=foundation.enum.numPorts2.two  m_specify=off  m_priority=High  m=1 kg  m_nominal_specify=off  m_nominal_value=1  m_nominal_unit=kg  T_specify=on  T_priority=High  T=23 degC  T_nominal_specify=off  T_nominal_value=1  T_nominal_unit=K  Q_specify=off  Q_priority=None  Q=0 W  Q_nominal_specify=off  Q_nominal_value=1  Q_nominal_unit=W
      settings: InternalSimscapePortConfiguration="{\"Bottom\":[],\"Left\":[{\"id\":\"M\",\"label\":\"\",\"type\":\"foundation.thermal.thermal\"}],\"Right\":[{\"id\":\"N\",\"label\":\"\",\"type\":\"foundation.thermal.thermal\"}],\"Top\":[]}"
  Thermal Reference : fl_lib/Thermal/Thermal Elements/Thermal Reference
  Conn2 : PMIOPort  Side=Left
  Conn1 : PMIOPort  Port=2  Side=Right
  wires:
  Step/1 -> Simulink-PS Converter/1
  connections:
  Conn2/RConn1 -- Pipe (TL)3/RConn1
  Pipe (TL)3/LConn1 -- Conn1/RConn1
  Simulink-PS Converter/RConn1 -- Controlled Heat Flow Rate Source/RConn1
  Thermal Reference/LConn1 -- Controlled Heat Flow Rate Source/RConn2
  Thermal Mass/LConn1 -- Pipe (TL)3/LConn2
  Thermal Mass/RConn1 -- Controlled Heat Flow Rate Source/LConn1

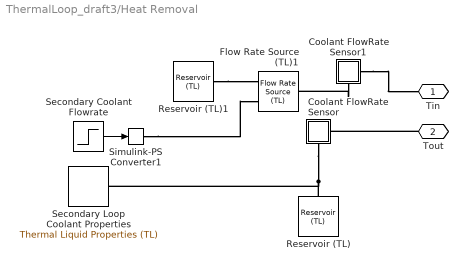
== system ThermalLoop_draft3/Heat Removal ==
  Coolant FlowRate Sensor : Subsystem
      settings: PortSchema="{\"entries\":[{\"content\":{\"sides\":[{\"content\":{\"connectorIds\":[\"LConn1\"]},\"type\":\"ConnectorPlacement.EquallySpacedRectSide\",\"uuid\":\"6f089a74-6670-43a9-89ac-660024aed54b\"},{\"content\":{\"side\":\"RIGHT\"},\"type\":\"ConnectorPlacement.EquallySpacedRectSide\",\"uuid\":\"d542e1c8-a7bd-4ccf-beed-7400ae0284ce\"},{\"content\":{\"side\":\"TOP\"},\"type\":\"ConnectorPlacement.EquallySpacedRectSide\",\"uuid\":\"3263a71e-8a0f-405c-8bee-b6e0c0a4cf43\"},{\"content\":{\"connectorIds\":[\"RConn1\"],\"side\":\"BOTTOM\"},\"type\":\"ConnectorPlacement.EquallySpacedRectSide\",\"uuid\":\"f84c467f-601c-45c8-b4c1-4a11ac0dd09f\"}]},\"type\":\"ConnectorPlacement.EquallySpacedConnector\",\"uuid\":\"c50b1cc5-df45-4c36-a930-71fffc74c8a0\"}],\"packageUris\":[\"http://schema.mathworks.com/mf0/Connector/R2020b\"],\"version\":\"1.0\"}"
  Coolant FlowRate Sensor1 : Subsystem
      settings: PortSchema="{\"entries\":[{\"content\":{\"sides\":[{\"content\":{\"connectorIds\":[\"LConn1\"]},\"type\":\"ConnectorPlacement.EquallySpacedRectSide\",\"uuid\":\"6f089a74-6670-43a9-89ac-660024aed54b\"},{\"content\":{\"side\":\"RIGHT\"},\"type\":\"ConnectorPlacement.EquallySpacedRectSide\",\"uuid\":\"d542e1c8-a7bd-4ccf-beed-7400ae0284ce\"},{\"content\":{\"side\":\"TOP\"},\"type\":\"ConnectorPlacement.EquallySpacedRectSide\",\"uuid\":\"3263a71e-8a0f-405c-8bee-b6e0c0a4cf43\"},{\"content\":{\"connectorIds\":[\"RConn1\"],\"side\":\"BOTTOM\"},\"type\":\"ConnectorPlacement.EquallySpacedRectSide\",\"uuid\":\"f84c467f-601c-45c8-b4c1-4a11ac0dd09f\"}]},\"type\":\"ConnectorPlacement.EquallySpacedConnector\",\"uuid\":\"c50b1cc5-df45-4c36-a930-71fffc74c8a0\"}],\"packageUris\":[\"http://schema.mathworks.com/mf0/Connector/R2020b\"],\"version\":\"1.0\"}"
  Flow Rate Source (TL)1 : fl_lib/Thermal Liquid/Sources/Flow Rate Source (TL)  source_type=foundation.enum.constant_controlled.controlled  flow_type=foundation.enum.mass_volumetric_flow.volumetric  mass_flow=0 kg/s  volumetric_flow=0 m^3/s  power_spec=foundation.enum.power_spec.isentropic  area=0.196 in^2
      settings: InternalSimscapePortConfiguration="{\"Bottom\":[],\"Left\":[{\"id\":\"A\",\"label\":\"A\",\"type\":\"foundation.thermal_liquid.thermal_liquid\"},{\"id\":\"V\",\"label\":\"V\",\"type\":\"input\"}],\"Right\":[{\"id\":\"B\",\"label\":\"B\",\"type\":\"foundation.thermal_liquid.thermal_liquid\"}],\"Top\":[]}"
  Reservoir (TL) : fl_lib/Thermal Liquid/Elements/Reservoir (TL)  pressure_spec=foundation.enum.pressure_spec.atmospheric  reservoir_pressure=0.101325 MPa  reservoir_temperature=297.15 K  area=0.441 in^2
  Reservoir (TL)1 : fl_lib/Thermal Liquid/Elements/Reservoir (TL)  pressure_spec=foundation.enum.pressure_spec.atmospheric  reservoir_pressure=0.101325 MPa  reservoir_temperature=19.6 degC  area=0.441 m^2
  Secondary Coolant Flowrate : Step  SampleTime=0
  Secondary Loop Coolant Properties : SimscapeFluids_lib/Thermal Liquid/Utilities/Thermal Liquid Properties (TL)  fluid_list=fluids.thermal_liquid.utilities.enum.thermal_liquid_fluid_list.water  concentration_param_EG=fluids.thermal_liquid.utilities.enum.thermal_liquid_concentration.volume_fraction  concentration_param_PG=fluids.thermal_liquid.utilities.enum.thermal_liquid_concentration.volume_fraction  c_mass_SW=3.5e-3  c_mass_EG=0.1  c_mass_PG=0.1  c_mass_GL=0.1  c_vol_EG=0.1  c_vol_PG=0.1  beta_const_EG=2.1791 GPa  beta_const_PG=2.1791 GPa  beta_const_GL=2.1791 GPa  p_min_EG=0.01 MPa  p_min_PG=0.01 MPa  p_min_GL=0.01 MPa  p_max_EG=50 MPa  p_max_PG=50 MPa  p_max_GL=50 MPa  p_atm=0.101325 MPa  properties_range_check=simscape.enum.assert.action.error
  Simulink-PS Converter1 : nesl_utility/Simulink-PS Converter  PhysicalDomain=network_engine_domain  SubClassName=ps_input  LeftPortType=input  RightPortType=output  PseudoPeriodic=off  Frequencies=[]  NoiseDistribution=none  NoiseParameters=[]  Unit=gpm  AffineConversion=off  FilteringAndDerivatives=provide  SimscapeFilterOrder=1  InputFilterTimeConstant=0.001  UdotUserProvided=0
  Tin : PMIOPort  Side=Right
  Tout : PMIOPort  Port=2  Side=Right
  wires:
  Secondary Coolant Flowrate/1 -> Simulink-PS Converter1/1
  connections:
  Reservoir (TL)/LConn1 -- Coolant FlowRate Sensor/RConn1 -- Secondary Loop Coolant Properties/RConn1
  Tout/RConn1 -- Coolant FlowRate Sensor/LConn1
  Reservoir (TL)1/LConn1 -- Flow Rate Source (TL)1/LConn1
  Simulink-PS Converter1/RConn1 -- Flow Rate Source (TL)1/LConn2
  Coolant FlowRate Sensor1/LConn1 -- Tin/RConn1
  Coolant FlowRate Sensor1/RConn1 -- Flow Rate Source (TL)1/RConn1
